simulink model "ECG_Rhythm_PVC_Detection_v4HighF_"  (R2019a)
settings: Solver=FixedStepDiscrete  StartTime=0.0  StopTime=10  FixedStep=1/360  RelTol=1e-3
libraries: simulink x13, dspstat3 x5, dspfdesign x2
settings Model: Creator=atif  LastModifiedBy=Admin
settings HardwareCC: ProdHWDeviceType=AMD->x86-64 (Windows64)

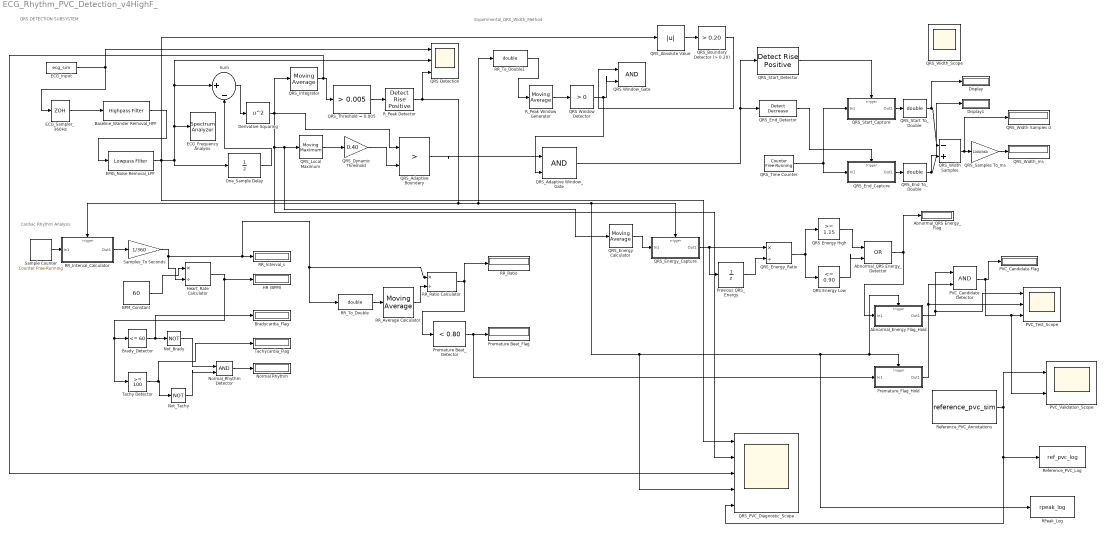
== system ECG_Rhythm_PVC_Detection_v4HighF_ ==
  note: Experimental_QRS_Width_Method
  note: Cardiac Rhythm Analysis
  note: QRS DETECTION SUBSYSTEM
  Abnormal_Energy Flag_Hold : Subsystem  TreatAsAtomicUnit=on
  Abnormal_QRS Energy_Detector : Logic  Operator=OR  IconShape=distinctive  AllPortsSameDT=off  OutDataTypeStr=boolean
  Abnormal_QRS Energy_Flag : Display
  BPM_Constant : Constant  Value=60
  Baseline_Wander Removal_HPF : dspfdesign/Highpass Filter  FilterType=FIR  DesignForMinimumOrder=on  FilterOrder=50  StopbandFrequency=0.1  PassbandFrequency=0.5  StopbandAttenuation=80  PassbandRipple=0.1  InheritSampleRate=off  SampleRate=360  SimulateUsing=Interpreted execution  roundingMode=Floor  coeffsDataTypeStr=fixdt(1,16)
      settings: SourceProductName=DSP System Toolbox
  Brady_Detector : simulink/Logic and Bit Operations/Compare To Constant  relop=<=  const=60  OutDataTypeStr=boolean
  Bradycardia_Flag : Display
  Derivative Squaring : Math  Operator=square  SaturateOnIntegerOverflow=on
  Display : Display
  Display1 : Display
  ECG_Frequency Analysis : SpectrumAnalyzer
  ECG_Input : FromWorkspace  VariableName=ecg_sim  SampleTime=0  Interpolate=off  OutputAfterFinalValue=Holding final value
  ECG_Sampler_360Hz : ZeroOrderHold  SampleTime=1/360
  EMG_Noise Removal_LPF : dspfdesign/Lowpass Filter  FilterType=FIR  DesignForMinimumOrder=on  FilterOrder=50  PassbandFrequency=40  StopbandFrequency=45  PassbandRipple=0.1  StopbandAttenuation=80  InheritSampleRate=off  SampleRate=360  SimulateUsing=Interpreted execution  roundingMode=Floor  coeffsDataTypeStr=fixdt(1,16)
  HR (BPM) : Display
  Heart_Rate Calculator : Product  Inputs=*/
  Normal Rhythm : Display
  Normal_Rhythm Detector : Logic  IconShape=distinctive  AllPortsSameDT=off  OutDataTypeStr=boolean
  Not_Brady : Logic  Operator=NOT  IconShape=distinctive  AllPortsSameDT=off  OutDataTypeStr=boolean
  Not_Tachy : Logic  Operator=NOT  IconShape=distinctive  AllPortsSameDT=off  OutDataTypeStr=boolean
  One_Sample Delay : UnitDelay  SampleTime=1/360  HasFrameUpgradeWarning=on
  PVC_Candidate Detector : Logic  AllPortsSameDT=off  OutDataTypeStr=boolean
  PVC_Candidate Flag : Display
  PVC_Test_Scope : Scope  NumInputPorts=3
  PVC_Validation_Scope : Scope  NumInputPorts=2
  Premature Beat_Detector : simulink/Logic and Bit Operations/Compare To Constant  relop=<  const=0.80  OutDataTypeStr=boolean
  Premature Beat_Flag : Display
  Premature_Flag_Hold : Subsystem  TreatAsAtomicUnit=on
  Previous QRS_Energy : UnitDelay  SampleTime=-1  HasFrameUpgradeWarning=on
  QRS Energy High : simulink/Logic and Bit Operations/Compare To Constant  relop=>=  const=1.15  OutDataTypeStr=boolean
  QRS Energy Low : simulink/Logic and Bit Operations/Compare To Constant  relop=<=  const=0.90  OutDataTypeStr=boolean
  QRS Window Detector : simulink/Logic and Bit Operations/Compare To Constant  relop=>  const=0  OutDataTypeStr=boolean
  QRS Window_Gate : Logic  IconShape=distinctive  AllPortsSameDT=off  OutDataTypeStr=boolean
  QRS Detection : Scope  NumInputPorts=3
  QRS_Absolute Value : Abs
  QRS_Adaptive Boundary : RelationalOperator  Operator=>  OutDataTypeStr=boolean  RndMeth=Simplest
  QRS_Adaptive Window_Gate : Logic  IconShape=distinctive  AllPortsSameDT=off  OutDataTypeStr=boolean
  QRS_Boundary Detector (> 0.20) : simulink/Logic and Bit Operations/Compare To Constant  relop=>  const=0.20  OutDataTypeStr=boolean
  "QRS_Dynamic Threshold " : Gain  Gain=0.40
  QRS_End To_Double : DataTypeConversion  OutDataTypeStr=double
  QRS_End_Capture : Subsystem  TreatAsAtomicUnit=on
  QRS_End_Detector : simulink/Logic and Bit Operations/Detect Decrease  vinit=0.0  OutDataTypeStr=boolean
  QRS_Energy Calculator : dspstat3/Moving Average  Method=Sliding window  ForgettingFactorPort=off  SpecifyWindowLength=on  WindowLength=54  ForgettingFactor=0.9  SimulateUsing=Code generation
  QRS_Energy_Capture : Subsystem  TreatAsAtomicUnit=on
  "QRS_Energy_Ratio " : Product  Inputs=*/
  QRS_Integrator : dspstat3/Moving Average  Method=Sliding window  ForgettingFactorPort=off  SpecifyWindowLength=on  WindowLength=54  ForgettingFactor=0.9  SimulateUsing=Code generation
  QRS_Local Maximum : dspstat3/Moving Maximum  SpecifyWindowLength=on  WindowLength=36  SimulateUsing=Code generation
      settings: SourceProductName=DSP System Toolbox  SourceProductBaseCode=DS
  QRS_PVC_Diagnostic_Scope : Scope  NumInputPorts=5
  QRS_Samples To_ms : Gain  Gain=1000/360
  QRS_Start To_Double : DataTypeConversion  OutDataTypeStr=double
  QRS_Start_Capture : Subsystem  TreatAsAtomicUnit=on
  QRS_Start_Detector : simulink/Logic and Bit Operations/Detect Rise Positive  vinit=0  OutDataTypeStr=boolean
  QRS_Threshold = 0.005 : simulink/Logic and Bit Operations/Compare To Constant  relop=>  const=0.005  OutDataTypeStr=boolean
  QRS_Time Counter : simulink/Sources/Counter Free-Running  NumBits=32  tsamp=1/360
  QRS_Width Samples : Sum  Inputs=-+
  QRS_Width Samples d : Display
  QRS_Width_Scope : Scope
  QRS_Width_ms : Display
  RPeak_Log : ToWorkspace  VariableName=rpeak_log  SaveFormat=Structure With Time  SampleTime=-1
  RR_Average Calculator : dspstat3/Moving Average  Method=Sliding window  ForgettingFactorPort=off  SpecifyWindowLength=on  WindowLength=8  ForgettingFactor=0.9  SimulateUsing=Code generation
  RR_Interval_Calculator : Subsystem  TreatAsAtomicUnit=on
  RR_Interval_s : Display
  RR_Ratio : Display
  RR_Ratio Calculator : Product  Inputs=*/
  RR_To_Double : DataTypeConversion  OutDataTypeStr=double
  RR_To_Double1 : DataTypeConversion  OutDataTypeStr=double
  R_Peak Detector : simulink/Logic and Bit Operations/Detect Rise Positive  vinit=0  OutDataTypeStr=boolean
  R_Peak Window Generator : dspstat3/Moving Average  Method=Sliding window  ForgettingFactorPort=off  SpecifyWindowLength=on  WindowLength=54  ForgettingFactor=0.9  SimulateUsing=Code generation
  Reference_PVC_Annotations : FromWorkspace  VariableName=reference_pvc_sim  SampleTime=0
  Reference_PVC_Log : ToWorkspace  VariableName=ref_pvc_log  SaveFormat=Structure With Time  SampleTime=-1
  Sample Counter : simulink/Sources/Counter Free-Running  NumBits=32  tsamp=1/360
  Samples_To Seconds : Gain  Gain=1/360
  Sum : Sum  Inputs=|+-
  Tachy Detector : simulink/Logic and Bit Operations/Compare To Constant  relop=>=  const=100  OutDataTypeStr=boolean
  Tachycardia_Flag : Display
  wires:
  ECG_Input/1 -> ECG_Sampler_360Hz/1, QRS Detection/1
  Baseline_Wander Removal_HPF/1 -> EMG_Noise Removal_LPF/1
  ECG_Sampler_360Hz/1 -> Baseline_Wander Removal_HPF/1
  One_Sample Delay/1 -> Sum/2
  EMG_Noise Removal_LPF/1 -> QRS_PVC_Diagnostic_Scope/1, QRS_Absolute Value/1, QRS Detection/2, Sum/1, ECG_Frequency Analysis/1, One_Sample Delay/1
  Sum/1 -> Derivative Squaring/1
  QRS_Integrator/1 -> QRS_PVC_Diagnostic_Scope/3, QRS_Threshold = 0.005/1
  Derivative Squaring/1 -> QRS_PVC_Diagnostic_Scope/2, QRS_Energy Calculator/1, QRS_Local Maximum/1, QRS_Adaptive Boundary/1, QRS_Integrator/1
  QRS_Threshold = 0.005/1 -> R_Peak Detector/1
  Sample Counter/1 -> RR_Interval_Calculator/1(In1)
  RR_Interval_Calculator/1(Out1) -> Samples_To Seconds/1
  Samples_To Seconds/1 -> RR_To_Double/1, RR_Ratio Calculator/1, RR_Interval_s/1, Heart_Rate Calculator/2
  BPM_Constant/1 -> Heart_Rate Calculator/1
  Heart_Rate Calculator/1 -> Tachy Detector/1, Brady_Detector/1, HR (BPM)/1
  Brady_Detector/1 -> Bradycardia_Flag/1, Not_Brady/1
  Tachy Detector/1 -> Not_Tachy/1, Tachycardia_Flag/1
  Not_Tachy/1 -> Normal_Rhythm Detector/2
  Not_Brady/1 -> Normal_Rhythm Detector/1
  Normal_Rhythm Detector/1 -> Normal Rhythm/1
  RR_Average Calculator/1 -> RR_Ratio Calculator/2
  RR_Ratio Calculator/1 -> RR_Ratio/1, Premature Beat_Detector/1
  RR_To_Double/1 -> RR_Average Calculator/1
  Premature Beat_Detector/1 -> Premature_Flag_Hold/1(In1), Premature Beat_Flag/1
  QRS_Absolute Value/1 -> QRS_Boundary Detector (> 0.20)/1
  QRS_Boundary Detector (> 0.20)/1 -> QRS Window_Gate/1
  QRS_Start_Detector/1 -> QRS_Start_Capture/Trigger
  QRS_Time Counter/1 -> QRS_End_Capture/1(In1), QRS_Start_Capture/1(In1)
  QRS_End_Detector/1 -> QRS_End_Capture/Trigger
  QRS_Start_Capture/1(Out1) -> QRS_Start To_Double/1
  QRS_Start To_Double/1 -> Display/1, QRS_Width Samples/1
  QRS_End_Capture/1(Out1) -> QRS_End To_Double/1
  QRS_End To_Double/1 -> Display1/1, QRS_Width Samples/2
  QRS_Width Samples/1 -> QRS_Width Samples d/1, QRS_Samples To_ms/1
  QRS_Samples To_ms/1 -> QRS_Width_ms/1
  R_Peak Window Generator/1 -> QRS Window Detector/1
  RR_To_Double1/1 -> R_Peak Window Generator/1
  QRS Window Detector/1 -> QRS_Adaptive Window_Gate/2, QRS Window_Gate/2
  QRS_Local Maximum/1 -> "QRS_Dynamic Threshold "/1
  "QRS_Dynamic Threshold "/1 -> QRS_Adaptive Boundary/2
  QRS_Adaptive Boundary/1 -> QRS_Adaptive Window_Gate/1
  QRS_Adaptive Window_Gate/1 -> QRS_End_Detector/1, QRS_Start_Detector/1
  QRS_Energy Calculator/1 -> QRS_Energy_Capture/1(In1)
  QRS_Energy_Capture/1(Out1) -> "QRS_Energy_Ratio "/1, Previous QRS_Energy/1
  Previous QRS_Energy/1 -> "QRS_Energy_Ratio "/2
  "QRS_Energy_Ratio "/1 -> QRS Energy Low/1, QRS Energy High/1
  QRS Energy High/1 -> Abnormal_QRS Energy_Detector/1
  QRS Energy Low/1 -> Abnormal_QRS Energy_Detector/2
  Abnormal_QRS Energy_Detector/1 -> Abnormal_QRS Energy_Flag/1, Abnormal_Energy Flag_Hold/1(In1)
  PVC_Candidate Detector/1 -> PVC_Validation_Scope/2, PVC_Test_Scope/3, PVC_Candidate Flag/1
  Abnormal_Energy Flag_Hold/1(Out1) -> PVC_Candidate Detector/1, PVC_Test_Scope/1
  Premature_Flag_Hold/1(Out1) -> PVC_Test_Scope/2, PVC_Candidate Detector/2
  Reference_PVC_Annotations/1 -> QRS_PVC_Diagnostic_Scope/5, Reference_PVC_Log/1, PVC_Validation_Scope/1
  R_Peak Detector/1 -> QRS Detection/3, QRS_PVC_Diagnostic_Scope/4, RPeak_Log/1, Premature_Flag_Hold/Trigger, Abnormal_Energy Flag_Hold/Trigger, QRS_Energy_Capture/Trigger, RR_To_Double1/1, RR_Interval_Calculator/Trigger

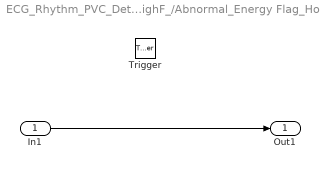
== system ECG_Rhythm_PVC_Detection_v4HighF_/Abnormal_Energy Flag_Hold ==
  In1 : Inport
  Trigger : TriggerPort  VariantControl=Variant
  Out1 : Outport
  wires:
  In1/1 -> Out1/1

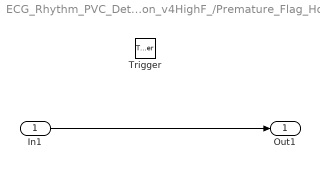
== system ECG_Rhythm_PVC_Detection_v4HighF_/Premature_Flag_Hold ==
  In1 : Inport
  Trigger : TriggerPort  VariantControl=Variant
  Out1 : Outport
  wires:
  In1/1 -> Out1/1

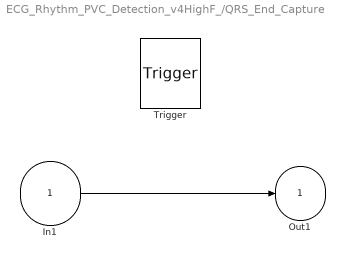
== system ECG_Rhythm_PVC_Detection_v4HighF_/QRS_End_Capture ==
  In1 : Inport
  Trigger : TriggerPort  VariantControl=Variant
  Out1 : Outport
  wires:
  In1/1 -> Out1/1

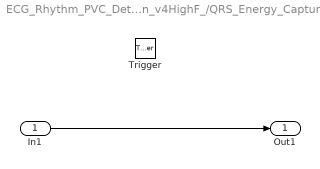
== system ECG_Rhythm_PVC_Detection_v4HighF_/QRS_Energy_Capture ==
  In1 : Inport
  Trigger : TriggerPort  VariantControl=Variant
  Out1 : Outport
  wires:
  In1/1 -> Out1/1

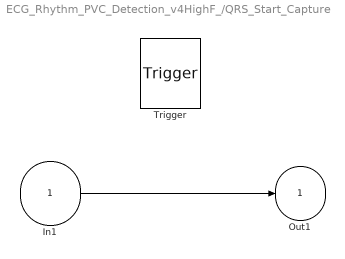
== system ECG_Rhythm_PVC_Detection_v4HighF_/QRS_Start_Capture ==
  In1 : Inport
  Trigger : TriggerPort  VariantControl=Variant
  Out1 : Outport
  wires:
  In1/1 -> Out1/1

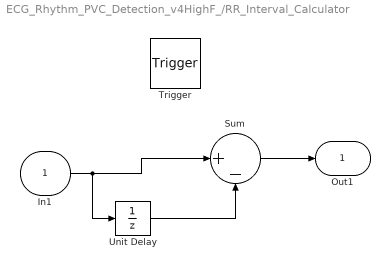
== system ECG_Rhythm_PVC_Detection_v4HighF_/RR_Interval_Calculator ==
  In1 : Inport
  Trigger : TriggerPort  VariantControl=Variant
  Sum : Sum  Inputs=|+-
  Unit Delay : UnitDelay  SampleTime=-1  HasFrameUpgradeWarning=on
  Out1 : Outport
  wires:
  In1/1 -> Unit Delay/1, Sum/1
  Unit Delay/1 -> Sum/2
  Sum/1 -> Out1/1
